simulink model "Project2_Sim_V2"  (R2019a)
settings: Solver=VariableStepAuto  StartTime=0.0  StopTime=tf  RelTol=1e-3
values from neighbouring files (symbols this model uses):
  a0 = [0;0;0]    [Project2_Main_V2.m]
  delta = [U(3);U(4);U(5);U(6)]    [FT_Quad.m]    (also in Project2_Main_V2.m = delta_yaw)
  g = U(11)    [FT_Quad.m]    (also in Forces_torques.m = 9.8; Project2_Main_V2.m = 9.8)
  J = [Jx;Jy;Jz]    [MomentsofInertia.m]    (also in Project2_Main_V2.m = MomentsofInertia([M,R,m,l]))
  k1 = U(7)    [FT_Quad.m]    (also in Project2_Main_V2.m = 1)
  k2 = U(8)    [FT_Quad.m]    (also in Project2_Main_V2.m = 0.75)
  l = U(9)    [FT_Quad.m]    (also in MomentsofInertia.m = U(4); Project2_Main_V2.m = 0.2)
  mt = M+4*m    (= 0.29)    [Project2_Main_V2.m]
  vel_initial = [v0;da0]    [Project2_Main_V2.m]
  x0 = [0;0;10]    [Project2_Main_V2.m]
undefined symbols (not defined in the file or in its folder): dynamics, FT_Quad, Rotational_Kinematic, Trans_Kinematic
settings Model: Creator=Andrew  LastModifiedBy=Andrew

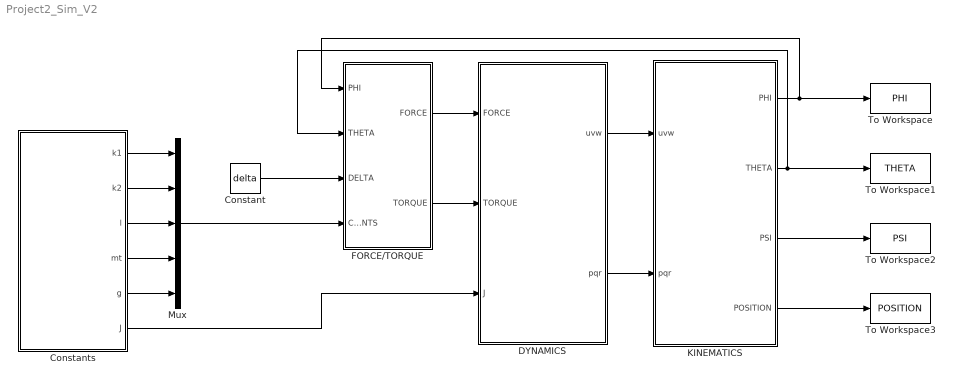
== system Project2_Sim_V2 ==
  Constant : Constant  Value=delta
  Constants : Subsystem
  DYNAMICS : Subsystem
  FORCE/TORQUE : Subsystem
  KINEMATICS : Subsystem
  Mux : Mux  Inputs=5
  To Workspace : ToWorkspace  VariableName=PHI  SaveFormat=Timeseries  SampleTime=-1
  To Workspace1 : ToWorkspace  VariableName=THETA  SaveFormat=Timeseries  SampleTime=-1
  To Workspace2 : ToWorkspace  VariableName=PSI  SaveFormat=Timeseries  SampleTime=-1
  To Workspace3 : ToWorkspace  VariableName=POSITION  SaveFormat=Timeseries  SampleTime=-1
  wires:
  Constants/1(k1) -> Mux/1
  Constants/2(k2) -> Mux/2
  Constants/3(l) -> Mux/3
  Constants/4(mt) -> Mux/4
  Constants/5(g) -> Mux/5
  Mux/1 -> FORCE/TORQUE/4(CONSTANTS)
  Constant/1 -> FORCE/TORQUE/3(DELTA)
  FORCE/TORQUE/1(FORCE) -> DYNAMICS/1(FORCE)
  FORCE/TORQUE/2(TORQUE) -> DYNAMICS/2(TORQUE)
  Constants/6(J) -> DYNAMICS/3(J)
  DYNAMICS/2(pqr) -> KINEMATICS/2(pqr)
  DYNAMICS/1(uvw) -> KINEMATICS/1(uvw)
  KINEMATICS/1(PHI) -> To Workspace/1, FORCE/TORQUE/1(PHI)
  KINEMATICS/2(THETA) -> To Workspace1/1, FORCE/TORQUE/2(THETA)
  KINEMATICS/4(POSITION) -> To Workspace3/1
  KINEMATICS/3(PSI) -> To Workspace2/1

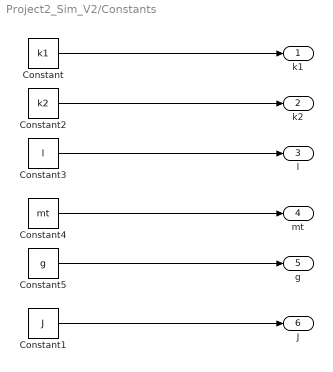
== system Project2_Sim_V2/Constants ==
  Constant : Constant  Value=k1
  Constant1 : Constant  Value=J
  Constant2 : Constant  Value=k2
  Constant3 : Constant  Value=l
  Constant4 : Constant  Value=mt
  Constant5 : Constant  Value=g
  k1 : Outport
  k2 : Outport  Port=2
  l : Outport  Port=3
  mt : Outport  Port=4
  g : Outport  Port=5
  J : Outport  Port=6
  wires:
  Constant/1 -> k1/1
  Constant2/1 -> k2/1
  Constant3/1 -> l/1
  Constant4/1 -> mt/1
  Constant5/1 -> g/1
  Constant1/1 -> J/1

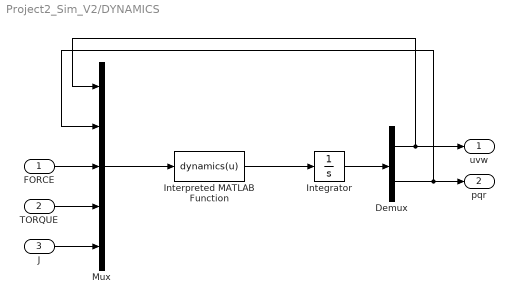
== system Project2_Sim_V2/DYNAMICS ==
  FORCE : Inport
  TORQUE : Inport  Port=2
  J : Inport  Port=3
  Demux : Demux  Outputs=2
  Integrator : Integrator  InitialCondition=vel_initial
  Interpreted MATLAB Function : MATLABFcn  MATLABFcn=dynamics(u)
  Mux : Mux  Inputs=[3;3;3;3;3]
  uvw : Outport
  pqr : Outport  Port=2
  wires:
  Interpreted MATLAB Function/1 -> Integrator/1
  J/1 -> Mux/5
  TORQUE/1 -> Mux/4
  FORCE/1 -> Mux/3
  Mux/1 -> Interpreted MATLAB Function/1
  Integrator/1 -> Demux/1
  Demux/1 -> Mux/1, uvw/1
  Demux/2 -> Mux/2, pqr/1

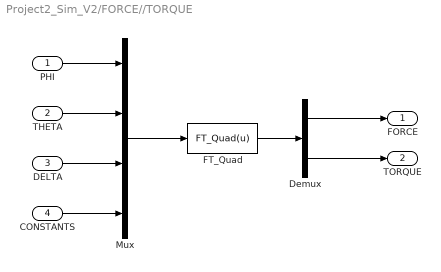
== system Project2_Sim_V2/FORCE//TORQUE ==
  PHI : Inport
  THETA : Inport  Port=2
  DELTA : Inport  Port=3
  CONSTANTS : Inport  Port=4
  Demux : Demux  Outputs=[3;3]
  FT_Quad : MATLABFcn  MATLABFcn=FT_Quad(u)
  Mux : Mux  Inputs=[1;1;4;5]
  FORCE : Outport
  TORQUE : Outport  Port=2
  wires:
  PHI/1 -> Mux/1
  THETA/1 -> Mux/2
  DELTA/1 -> Mux/3
  CONSTANTS/1 -> Mux/4
  Mux/1 -> FT_Quad/1
  FT_Quad/1 -> Demux/1
  Demux/1 -> FORCE/1
  Demux/2 -> TORQUE/1

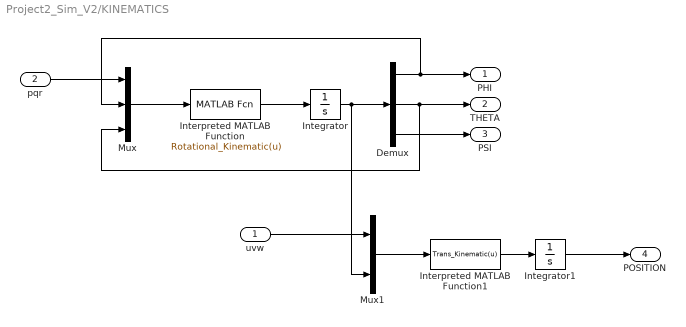
== system Project2_Sim_V2/KINEMATICS ==
  uvw : Inport
  pqr : Inport  Port=2
  Demux : Demux  Outputs=3
  Integrator : Integrator  InitialCondition=a0
  Integrator1 : Integrator  InitialCondition=x0
  Interpreted MATLAB Function : MATLABFcn  MATLABFcn=Rotational_Kinematic(u)
  Interpreted MATLAB Function1 : MATLABFcn  MATLABFcn=Trans_Kinematic(u)
  Mux : Mux  Inputs=[3;1;1]
  Mux1 : Mux  Inputs=[3;3]
  PHI : Outport
  THETA : Outport  Port=2
  PSI : Outport  Port=3
  POSITION : Outport  Port=4
  wires:
  pqr/1 -> Mux/1
  Mux/1 -> Interpreted MATLAB Function/1
  Interpreted MATLAB Function/1 -> Integrator/1
  Integrator/1 -> Mux1/2, Demux/1
  Demux/1 -> Mux/2, PHI/1
  Demux/2 -> Mux/3, THETA/1
  Demux/3 -> PSI/1
  uvw/1 -> Mux1/1
  Mux1/1 -> Interpreted MATLAB Function1/1
  Interpreted MATLAB Function1/1 -> Integrator1/1
  Integrator1/1 -> POSITION/1
